simulink model "model"  (R2025b)
settings: Solver=ode15s  StartTime=0.0  StopTime=9.2  MaxStep=0.000005  RelTol=1e-12  AbsTol=1e-12
values from neighbouring files (symbols this model uses):
  C1_opt = 1250 * (1 + exp(45)) / (47 + 43*exp(45))    [init.m]
  C2_opt = -250 * (1 - exp(45)) / (47 + 43*exp(45))    [init.m]
  R = 5    [init.m]
  x1_0 = 0    [init.m]
  x2_0 = 0    [init.m]
settings Model: Creator=eva  LastModifiedBy=eva
settings SolverCC: AutoScaleAbsTol=off  SolverResetMethod=Robust

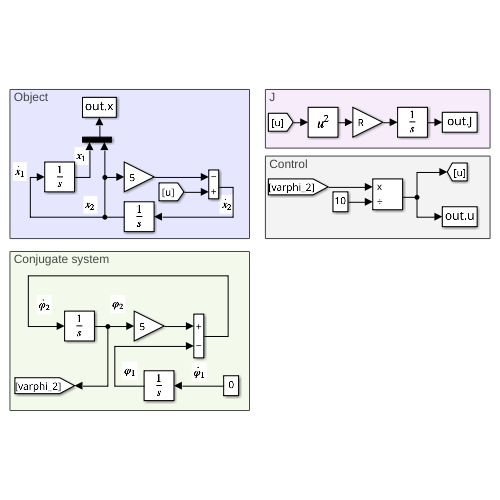
[thumbnail: Simulink's stored preview of the top-level diagram]
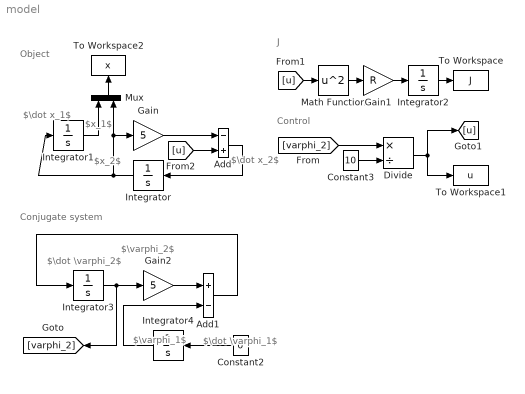
== system model ==
  note: Control
  note: Conjugate system
  note: J
  note: Object
  note: $\dot x_1$
  note: $x_1$
  note: $x_2$
  note: $\dot x_2$
  note: $\dot \varphi_2$
  note: $\varphi_2$
  note: $\dot \varphi_1$
  note: $\varphi_1$
  Add : Sum  Inputs=-+
  Add1 : Sum  Inputs=+-
  Constant2 : Constant  Value=0
  Constant3 : Constant  Value=10
  Divide : Product  Inputs=*/
  Gain : Gain  Gain=5
  Gain1 : Gain  Gain=R
  Gain2 : Gain  Gain=5
  Integrator : Integrator  InitialCondition=x2_0
  Integrator1 : Integrator  InitialCondition=x1_0
  Integrator2 : Integrator
  Integrator3 : Integrator  InitialCondition=C2_opt
  Integrator4 : Integrator  InitialCondition=C1_opt
  Math Function : Math  Operator=square
  Mux : Mux  Inputs=2
  To Workspace : ToWorkspace  VariableName=J  SaveFormat=Structure With Time  SampleTime=-1
  To Workspace1 : ToWorkspace  VariableName=u  SaveFormat=Structure With Time  SampleTime=-1
  To Workspace2 : ToWorkspace  VariableName=x  SaveFormat=Structure With Time  SampleTime=-1
  wires:
  Integrator/1 -> Integrator1/1, Mux/2, Gain/1
  Add/1 -> Integrator/1
  Integrator1/1 -> Mux/1
  [u] -> Add/2
  Gain/1 -> Add/1
  [u] -> Math Function/1
  Math Function/1 -> Gain1/1
  Gain1/1 -> Integrator2/1
  Integrator2/1 -> To Workspace/1
  Integrator3/1 -> [varphi_2], Gain2/1
  Constant2/1 -> Integrator4/1
  Gain2/1 -> Add1/1
  Add1/1 -> Integrator3/1
  [varphi_2] -> Divide/1
  Constant3/1 -> Divide/2
  Divide/1 -> [u], To Workspace1/1
  Integrator4/1 -> Add1/2
  Mux/1 -> To Workspace2/1
